simulink model "UAV_SIMULATOR_CA_2021a"  (R2024a)
settings: Solver=FixedStepAuto  StartTime=0.0  StopTime=tf_echelons  FixedStep=0.002  RelTol=1e-4
values from neighbouring files (symbols this model uses):
  Beta_OPT = [Beta, Z_max: 0.1*pi/180: betaf]    [UAV_SIMULATOR_MAIN_0.m]
  betaf = 20*pi/180 +betai    (= 0.660268528005)    [UAV_SIMULATOR_MAIN_0.m]
  betai = 17.8306*pi/180    (= 0.311202677606)    [UAV_SIMULATOR_MAIN_0.m]
  Bp_offset = 0.06    [UAV_SIMULATOR_MAIN_0.m]
  CDy = data(1)    [Aero_initial.m]    (also in FunLagragian.m; UAV_SIMULATOR_MAIN_0.m = 1; costFunction.m; nonLinearConstraints.m)
  CLOSED_LOOP_ESCs = 1    [UAV_SIMULATOR_MAIN_0.m]
  cQ = 2.1113*1e-08    (= 2.1113e-08)    [UAV_SIMULATOR_MAIN_0.m]
  cQ_Magnus = 0.5*S/2*RM^3*Cf    (= 4.804078125e-10)    [UAV_SIMULATOR_MAIN_0.m]
  cT = 2.4815e-6    (= 2.4815e-06)    [UAV_SIMULATOR_MAIN_0.m]
  cT_1_6 = 2.1030e-06    (= 2.103e-06)    [UAV_SIMULATOR_MAIN_0.m]
  D_PQR_PX4 = diag([D_ROLL D_PITCH D_YAW])    [UAV_SIMULATOR_MAIN_0.m]
  ethaf = 25*pi/180    (= 0.436332312999)    [UAV_SIMULATOR_MAIN_0.m]
  ethai = 0 *pi/180    (= 0)    [UAV_SIMULATOR_MAIN_0.m]
  F_fric = 0.5    [UAV_SIMULATOR_MAIN_0.m]
  Fa_L_int = Rmat*(FaG_int+FaG_int_d)    [UAV_SIMULATOR_MAIN_0.m]
  g = data(7)    [FunLagragian.m]    (also in UAV_SIMULATOR_MAIN_0.m = 9.81; costFunction.m; nonLinearConstraints.m; runOptimizationHelper.m = comp(7))
  I_PQR_PX4 = diag([I_ROLL I_PITCH I_YAW])    [UAV_SIMULATOR_MAIN_0.m]
  initial_attitude_condition = 1*[0 0 pi]    [UAV_SIMULATOR_MAIN_0.m]
  initial_pos_conditions = [ri*cos(betai) 0 ri*sin(betai) + Bp_offset]    [UAV_SIMULATOR_MAIN_0.m]
  Jr = 1.2991*1e-05    (= 1.2991e-05)    [UAV_SIMULATOR_MAIN_0.m]
  Jr_Magnus = JM1(2,2)    [UAV_SIMULATOR_MAIN_0.m]
  K_DI_int = [diag([k_r(1), k_etha(1), k_beta(1)]), diag([k_r(2), k_etha(2), k_beta(2)]), diag([k_r(3), k_etha(3), k_beta(3)])]    [UAV_SIMULATOR_MAIN_0.m]
  K_PQR_PX4 = 1*diag([0.8 1.35 1])    [UAV_SIMULATOR_MAIN_0.m]
  km = 1/Kv_motor_rad    (= 0.00545674090601)    [UAV_SIMULATOR_MAIN_0.m]
  L = lqr(A,B,Q_beta,R_beta)    [UAV_SIMULATOR_MAIN_0.m]
  L_mot = 1.0000e-04    (= 0.0001)    [UAV_SIMULATOR_MAIN_0.m]
  LM = 0.28*2    (= 0.56)    [UAV_SIMULATOR_MAIN_0.m]
  m = data(6)    [FunLagragian.m]    (also in UAV_SIMULATOR_MAIN_0.m = 1.746; costFunction.m; nonLinearConstraints.m; runOptimizationHelper.m = comp(6))
  m_M1 = 0.049    [UAV_SIMULATOR_MAIN_0.m]
  m_M2 = 0.049    [UAV_SIMULATOR_MAIN_0.m]
  m_w = 0.0481    [UAV_SIMULATOR_MAIN_0.m]    (also in nonLinearConstraints.m = data(9); runOptimizationHelper.m = comp(9))
  max_angle = max_angle_deg*pi/180    (= 0.610865238198)    [UAV_SIMULATOR_MAIN_0.m]
  nb_battery_cells = 4    [UAV_SIMULATOR_MAIN_0.m]
  P_ATTITUDE_PX4 = diag([10 10 2.8])    [UAV_SIMULATOR_MAIN_0.m]
  P_PQR_PX4 = diag([P_ROLL P_PITCH P_YAW])    [UAV_SIMULATOR_MAIN_0.m]
  PX4_attitude_loop_frequency = 250    [UAV_SIMULATOR_MAIN_0.m]
  PX4_rate_loop_frequency = 500    [UAV_SIMULATOR_MAIN_0.m]
  R = data(4)    [Aero_initial.m]    (also in UAV_SIMULATOR_MAIN_0.m = 0.07)
  R_bat = 0.024    [UAV_SIMULATOR_MAIN_0.m]
  rf = 1.5    [UAV_SIMULATOR_MAIN_0.m]
  rho_air = data(8)    [FunLagragian.m]    (also in UAV_SIMULATOR_MAIN_0.m = 1.293; costFunction.m; nonLinearConstraints.m; runOptimizationHelper.m = comp(8))
  ri = 0.490142    [UAV_SIMULATOR_MAIN_0.m]
  RM = data(4)    [FunLagragian.m]    (also in UAV_SIMULATOR_MAIN_0.m = 0.0275; costFunction.m; nonLinearConstraints.m; runOptimizationHelper.m = comp(4))
  S = data(3)    [Aero_initial.m]    (also in FunLagragian.m; UAV_SIMULATOR_MAIN_0.m = 0.0308; costFunction.m; nonLinearConstraints.m)
  s_M1D = [0, LM/4, 0]'    [UAV_SIMULATOR_MAIN_0.m]
  s_M2D = [0, -LM/4, 0]'    [UAV_SIMULATOR_MAIN_0.m]
  Slat = data(2)    [Aero_initial.m]    (also in FunLagragian.m; UAV_SIMULATOR_MAIN_0.m = 0.00237582944428; costFunction.m; nonLinearConstraints.m)
  state_int = [0 0 0 initial_attitude_condition 0 0 0 initial_attitude_quaternion_condition]    [UAV_SIMULATOR_MAIN_0.m]
  T0 = 1.5    [UAV_SIMULATOR_MAIN_0.m]
  t0 = 0    [UAV_SIMULATOR_MAIN_0.m]
  t1 = t0 + 15    (= 15)    [UAV_SIMULATOR_MAIN_0.m]
  t1T = t1/10    (= 1.5)    [UAV_SIMULATOR_MAIN_0.m]
  t2 = t1 + 15    (= 30)    [UAV_SIMULATOR_MAIN_0.m]    (also in plot_test.m = Simulation_Data.time)
  t2T = t2 + 9*t1/10    (= 43.5)    [UAV_SIMULATOR_MAIN_0.m]
  t3 = t2 + 15    (= 45)    [UAV_SIMULATOR_MAIN_0.m]
  tau_ur_model = 0.001    [UAV_SIMULATOR_MAIN_0.m]
  Tf = 1.5    [UAV_SIMULATOR_MAIN_0.m]
  Ti = 0    [UAV_SIMULATOR_MAIN_0.m]
  Ts = 0.02    [UAV_SIMULATOR_MAIN_0.m]
  U_sat = 3.7*nb_battery_cells    (= 14.8)    [UAV_SIMULATOR_MAIN_0.m]
  ViconTracker_noise_mean = 0.00001    (= 1e-05)    [UAV_SIMULATOR_MAIN_0.m]
  ViconTracker_noise_variance = 0.000001    (= 1e-06)    [UAV_SIMULATOR_MAIN_0.m]
  vitesse_vent = [0, 0, 0]'    [UAV_SIMULATOR_MAIN_0.m]
  vmag = 0    [UAV_SIMULATOR_MAIN_0.m]
  vx_wind = [vwind(1,1:t_winddirc_change/dt-1) vx_inter vwind(1,(t_winddirc_change+1)/dt +1:final_time/dt+1)*cos(10*pi/180)]    [UAV_SIMULATOR_MAIN_0.m]
  vy_wind = [zeros(1,t_winddirc_change/dt-1) vy_inter vwind(1,(t_winddirc_change+1)/dt +1:final_time/dt+1)*sin(10*pi/180)]    [UAV_SIMULATOR_MAIN_0.m]
  wind_turb = 1    [UAV_SIMULATOR_MAIN_0.m]
  wn_beta = 2    [UAV_SIMULATOR_MAIN_0.m]
  wn_etha = 2    [UAV_SIMULATOR_MAIN_0.m]
  wn_r = 2    [UAV_SIMULATOR_MAIN_0.m]
  X0 = 4    [UAV_SIMULATOR_MAIN_0.m]    (also in runOptimizationHelper.m = data(19))
  X1 = min(X1,8)    [Aero_initial.m]    (also in UAV_SIMULATOR_MAIN_0.m = [X1, X1(end)])
undefined symbols (not defined in the file or in its folder): DiscIntNeverNeededParam, PWM_data_map
libraries: simulink x23, slpidlib x5, eeGeneralControl x3, simulink_extras x1
(part 3 of 3)

== system UAV_SIMULATOR_CA_2021a/X4 + PX4 /X4 ESC PWM [OPEN LOOP MOTOR]1/Subsystem4/Subsystem2 ==
  In1 : Inport
  Gain4 : Gain  Gain=km
  Gain5 : Gain  Gain=km
  Gain6 : Gain  Gain=0.000001
  Gain7 : Gain  Gain=cQ
  Product1 : Product
  Sum3 : Sum  Inputs=|+-
  Sum4 : Sum  Inputs=-|+|-
  Transfer Fcn2 : TransferFcn  Denominator=[L_mot R]
  Transfer Fcn3 : TransferFcn  Denominator=[Jr 0]
  Out1 : Outport  VectorParamsAs1DForOutWhenUnconnected=off
  Out2 : Outport  Port=2  VectorParamsAs1DForOutWhenUnconnected=off
  wires:
  Sum4/1 -> Transfer Fcn3/1
  Gain5/1 -> Sum3/2  "FEM"
  Transfer Fcn3/1 -> Product1/2, Product1/1, Out1/1, Gain6/1, Gain5/1  "W"
  Gain4/1 -> Sum4/2  "Gama_mot"
  Product1/1 -> Gain7/1
  Gain6/1 -> Sum4/3  "Gamma_fric"
  Sum3/1 -> Transfer Fcn2/1
  Gain7/1 -> Sum4/1  "Gama_load"
  Transfer Fcn2/1 -> Out2/1, Gain4/1  "Motor_current"
  In1/1 -> Sum3/1  "U"

== system UAV_SIMULATOR_CA_2021a/X4 + PX4 /X4 ESC PWM [OPEN LOOP MOTOR]1/Subsystem4/Subsystem3 ==
  In1 : Inport
  Gain4 : Gain  Gain=km
  Gain5 : Gain  Gain=km
  Gain6 : Gain  Gain=0.000001
  Gain7 : Gain  Gain=cQ
  Product1 : Product
  Sum3 : Sum  Inputs=|+-
  Sum4 : Sum  Inputs=-|+|-
  Transfer Fcn2 : TransferFcn  Denominator=[L_mot R]
  Transfer Fcn3 : TransferFcn  Denominator=[Jr 0]
  Out1 : Outport  VectorParamsAs1DForOutWhenUnconnected=off
  Out2 : Outport  Port=2  VectorParamsAs1DForOutWhenUnconnected=off
  wires:
  In1/1 -> Sum3/1  "U"
  Transfer Fcn2/1 -> Gain4/1, Out2/1  "Motor_current"
  Gain7/1 -> Sum4/1  "Gama_load"
  Sum3/1 -> Transfer Fcn2/1
  Gain6/1 -> Sum4/3  "Gamma_fric"
  Product1/1 -> Gain7/1
  Gain4/1 -> Sum4/2  "Gama_mot"
  Transfer Fcn3/1 -> Gain5/1, Gain6/1, Out1/1, Product1/1, Product1/2  "W"
  Gain5/1 -> Sum3/2  "FEM"
  Sum4/1 -> Transfer Fcn3/1

== matlab function UAV_SIMULATOR_CA_2021a/spherical coordinates/MATLAB Function ==
  data: input input; spher_coord output
function  spher_coord = cart2spher(input)
x = input(1);
y = input(2);
z = input(3);
x_dot = input(4);
y_dot = input(5);
z_dot = input(6);

r = sqrt(x^2+y^2+z^2); %length of tether, [m]
if r > 0
    r_dir = -[x,y,z]./r; %unit vector of the tether [3x1] in inertial frame {I}
else
    r_dir = -[0,0,1];
end

xy=sqrt(x^2+y^2);
if xy ~= 0
  beta = atan2(z,xy);
  beta_dot = (xy*z_dot-z*(x*x_dot+y*y_dot)/xy)/r^2;
  etha_dot = (x*y_dot-y*x_dot)/(xy^2);
else
    beta = pi/2;
    etha_dot = 0;
    beta_dot = 0;
end


etha = atan2(y,x);
if r ~= 0
 r_dot = (x*x_dot+y*y_dot+z*z_dot)/r;
else
    r_dot = 0;
    beta_dot = 0;
end

spher_coord = [r etha beta r_dot etha_dot beta_dot r_dir];
spher_coord = double(spher_coord);
end

== matlab function UAV_SIMULATOR_CA_2021a/MATLAB Function6 ==
  data: input input; uT0_prev output
function uT0_prev = fcn(input)
Td=input(1);
r=input(2);
etha=input(3);
beta=input(4);
phi=input(5);
theta=input(6);
psi=input(7);
uT0_prev=Td*(cos(etha)*cos(beta)*cos(phi)*sin(theta)*cos(psi)+cos(etha)*cos(beta)*sin(phi)*sin(psi)+sin(etha)*cos(beta)*cos(phi)*sin(theta)*sin(psi)-sin(etha)*cos(beta)*sin(phi)*cos(psi)+sin(beta)*cos(phi)*cos(theta));
end

== matlab function UAV_SIMULATOR_CA_2021a/Subsystem2/MATLAB Function2 ==
  data: x_e input; xdot_e output; control input; data input
function xdot_e  = model_ekf(x_e,control, data)   % state : x_e =(r,dr,beta,dbeta,L,D)
m_w = data(1); 
m   = data(2); 
g   = data(3);

ur    = control(1);
uT    = control(2);
ubeta = control(3);
uetha = control(4);

xdot_e = [x_e(2);
         (1/(m+m_w))*(x_e(1)*x_e(6)^2*m +x_e(1)*x_e(4)^2*cos(x_e(5))^2*m -ur -m*g*sin(x_e(5))+uT + x_e(7));
         x_e(4);
         (1/(x_e(1)*cos(x_e(5))))*(-2*x_e(2)*x_e(4)*cos(x_e(5))+2*x_e(1)*x_e(4)*x_e(6)*sin(x_e(5))+1/m*uetha+1/m*x_e(8));
         x_e(6);
         (1/x_e(1))*(-2*x_e(2)*x_e(6)-x_e(1)*x_e(4)^2*cos(x_e(5))*sin(x_e(5))-g*cos(x_e(5))+1/m*ubeta + 1/m*x_e(9)); 
         0;
         0;
         0];
end

== matlab function UAV_SIMULATOR_CA_2021a/Subsystem2/Noice on Covariance ==
  data: u input; y output
function y = fcn(u)
y=randn*1e-4;
end

== matlab function UAV_SIMULATOR_CA_2021a/MATLAB Function2 ==
  data: Fa_G input; Fa_L output; data input
function Fa_L = fcn(Fa_G, data)
eta=data(2);
beta=data(3);
R_GS = [cos(eta)*cos(beta) sin(eta)*cos(beta) sin(beta);
                -sin(eta) cos(eta) 0;
                 -cos(eta)*sin(beta) -sin(eta)*sin(beta) cos(beta)];
Fa_L = R_GS * Fa_G;
end

== matlab function UAV_SIMULATOR_CA_2021a/MATLAB Function1 ==
  data: FaL input; u output; x input; data input
function u= fcn(FaL,x,data)
m = data(1);
m_w = data(2);
A = [(-1)/(m+m_w) 0 0;
    0 1/(m*x(1)*cos(x(3))) 0;
    0 0 1/(m*x(1))];
u = A * FaL;
end

== matlab function UAV_SIMULATOR_CA_2021a/2D LF Control3/CA optimisation problem1 ==
  settings: updateMethod=DISCRETE
  data: data input; optimized_X output; F_res_spherical output; Fa_zLB output; fval output; exitflag output; gradient output
function [optimized_X, F_res_spherical, Fa_zLB, fval, exitflag, gradient] = calculateOptimizedMagnusAndResidualForces(data)
% Wrapper that calls the full optimization helper (executed in MATLAB interpreter)

coder.extrinsic('runOptimizationHelper')

% Predefine output sizes and types
optimized_X = 0;
F_res_spherical = zeros(3,1);
Fa_zLB = 0;
fval = 0;
exitflag = int8(0);
gradient = 0;

% Call helper that performs all optimization and aerodynamic calculations
[optimized_X, F_res_spherical, Fa_zLB, fval, exitflag, gradient] = runOptimizationHelper(data);
end

== matlab function UAV_SIMULATOR_CA_2021a/MATLAB Function3 ==
  data: Fa_G input; Fa_L output; data input
function Fa_L = fcn(Fa_G, data)
eta=data(2);
beta=data(3);
R_GS = [cos(eta)*cos(beta) sin(eta)*cos(beta) sin(beta);
                -sin(eta) cos(eta) 0;
                 -cos(eta)*sin(beta) -sin(eta)*sin(beta) cos(beta)];
Fa_L = R_GS * Fa_G;
end

== matlab function UAV_SIMULATOR_CA_2021a/2D LF Control3/Compensation of F_res 1 ==
  data: pos_spherical input; F_res_spherical input; Fa_zLB input; thrust_ref output; phi_ref output; psi input; theta_ref output; psi_vicon input
function [thrust_ref, phi_ref, theta_ref] = calculateThrustAndPhi(pos_spherical, F_res_spherical, Fa_zLB, psi,psi_vicon)
    

    r    = pos_spherical(1);
    etha = pos_spherical(2);
    beta = pos_spherical(3);

    delta_FT    = F_res_spherical(1);
    delta_Feta  = F_res_spherical(2);
    delta_Fbeta = F_res_spherical(3);

    thrust_ref = norm(F_res_spherical);
    
    theta_ref = atan2((delta_FT*cos(etha)*cos(beta) - delta_Feta*sin(etha) - delta_Fbeta*cos(etha)*sin(beta)) * cos(psi+psi_vicon) +...
        (delta_FT*sin(etha)*cos(beta) + delta_Feta*cos(etha) - delta_Fbeta*sin(etha)*sin(beta)) * sin(psi+psi_vicon), (delta_FT*sin(beta) + delta_Fbeta*cos(beta)));

    T_dy = thrust_ref + Fa_zLB;%force acting on y direction
    if T_dy == 0  
      phi_ref = 0;
    else
      phi_ref = asin(((-delta_FT*sin(etha)*cos(beta) - delta_Feta*cos(etha) + delta_Fbeta*sin(etha)*sin(beta)) *cos(psi+psi_vicon) + ...
          (delta_FT*cos(etha)*cos(beta) - delta_Feta*sin(etha) - delta_Fbeta*cos(etha)*sin(beta)) * sin(psi+psi_vicon))/T_dy);
    end

%     theta_ref = atan2((delta_FT*cos(etha)*cos(beta) - delta_Feta*sin(etha) - delta_Fbeta*cos(etha)*sin(beta)) / cos(psi), (delta_FT*sin(beta) + delta_Fbeta*cos(beta)));
% 
%     T_dy = thrust_ref + Fa_zLB;%force acting on y direction
%     if T_dy == 0  
%       phi_ref = 0;
%     else
%       phi_ref = asin((-delta_FT*sin(etha)*cos(beta) - delta_Feta*cos(etha) + delta_Fbeta*sin(etha)*sin(beta)) /(T_dy*cos(psi)));
%     end
end

== matlab function UAV_SIMULATOR_CA_2021a/2D LF Control3/MATLAB Function ==
  data: input input; Va_G output
function Va_G = fcn(input)
V_wind = input(1:3);
V_system = input(4:6);
Va_G = V_wind - V_system;
end

== matlab function UAV_SIMULATOR_CA_2021a/2D LF Control3/MATLAB Function1 ==
  data: betaref input; BETA_OPT input; X1 input; X0 input; X_opt output
function X_opt  = fcn(betaref, BETA_OPT, X1, X0)
I=1;
while BETA_OPT(I)<=betaref && BETA_OPT(I)~=BETA_OPT(end)
    I=I+1;
end
X_opt=double(X1(I));
end

== matlab function UAV_SIMULATOR_CA_2021a/3D PID- open Loop uT/MATLAB Function ==
  data: input input; output output; psi input; max_roll_pitch input

function output = Thrust_phi_theta(input, psi, max_roll_pitch) 

Fx = input(1);
Fy = input(2);
Fz = input(3);


FX = cos(psi) * Fx  + sin(psi) * Fy;
FY = -sin(psi) * Fx + cos(psi) * Fy;


theta = atan2(FX,Fz);
if abs(theta) > max_roll_pitch
    theta = sign(theta) * max_roll_pitch;
    FX = Fz * tan(theta);
end
    
phi = atan2(-FY, sqrt(Fz^2+FX^2));
if abs(phi) > max_roll_pitch
   phi = sign(phi) * max_roll_pitch;
   FY = sqrt(Fz^2 + FX^2) * tan(phi);
end 
    

T_d = sqrt(FX^2 + FY^2 + Fz^2);  


T_ref = T_d;
phi_ref = phi;
theta_ref = theta;

output= [phi_ref,theta_ref, T_ref];
end

== matlab function UAV_SIMULATOR_CA_2021a/3D PID- open Loop uT/MATLAB Function1 ==
  settings: updateMethod=DISCRETE
  data: Trajectory_Error input; u_winch output; Integral_Error input; Derivative input; pos_speed_spher input; Feed_Forward input; data input; K_DI_int input; u_UAV output; data1 input; v output; ie_beta output; L input; T0 input; T_error input; T_error_int input
function [u_winch, u_UAV, v, ie_beta] = calculatePIDControlInput(Trajectory_Error,Integral_Error, Derivative, pos_speed_spher, Feed_Forward, data, K_DI_int,...
    data1, L, T0, T_error, T_error_int)

m_w = data(1);
wn_r = data(2);
wn_beta = data(3);
wn_etha = data(4);
m = data(5);    % mass of the total system
g = data(6);
%T0 = data(7);   % desired tether traction forc
betai = data(7); 
betaf = data(8);

v_beta_saturate_upper = 1.2;% m*g*cos(betai) + 0.1;
v_beta_saturate_lower = -0.1;% m*g*cos(max_angle) -0.1;


e_r    = Trajectory_Error(1);
e_etha = Trajectory_Error(2);
e_beta = Trajectory_Error(3);

de_r    = Trajectory_Error(4);
de_etha = Trajectory_Error(5);
de_beta = Trajectory_Error(6);

ie_r    = Integral_Error(1);
ie_etha = Integral_Error(2);
ie_beta = Integral_Error(3);

ddr    = Derivative(4);

r    = pos_speed_spher(1);
etha = pos_speed_spher(2);
beta = pos_speed_spher(3);

d_r    = pos_speed_spher(4);
d_etha = pos_speed_spher(5);
d_beta = pos_speed_spher(6);

% Feed Forward Terms
Fa_r    = Feed_Forward(1);
Fa_etha  = Feed_Forward(2);
Fa_beta = Feed_Forward(3);

if(r == 0)
    u_winch = 0;
    u_UAV = [0, 0, 0];
    v = [0, 0, 0]';
else
    
    
    %u_r_1 = 2*0.7*wn_r*de_r       + wn_r^2*e_r ;
    u_T = T0 + m*g*sin(beta);% + m*ddr;     % open loop on u_T 
   
    A = [-1/(m + m_w)      0               0;
            0       1/(m*r*cos(beta))      0;
            0              0            1/(m*r)];
        
    b=[(1/(m + m_w)) * ((r*d_beta^2 + r*d_etha^2*cos(beta)^2)*m - m*g*sin(beta) + u_T + Fa_r);
        
        (-2*d_r*d_etha*cos(beta) + 2*r*d_etha*d_beta*sin(beta) + (1/m) * Fa_etha)/(r*cos(beta));
        
        (-2*d_r*d_beta - r*d_etha^2*cos(beta)*sin(beta) - g*cos(beta) + (1/m)*Fa_beta)/r];

% Feedback Linearization based on PID + Anti windup 
    v_r    = 2.1396*wn_r*de_r       + 2.172*wn_r^2*e_r       + wn_r^3*ie_r;
    v_etha = 2.1396*wn_etha*de_etha  + 2.172*wn_etha^2*e_etha + wn_etha^3*ie_etha;
    v_beta = 2.1396*wn_beta*de_beta + 2.172*wn_beta^2*e_beta + wn_beta^3*ie_beta;
    
    
    % Feed back controller
    v=[v_r;v_etha;v_beta];
    u=A\(v-b);

    u_winch = u(1);
    %u_T = u_T + 1*max(1*(T0 - T) + 1*T_int,0);
    %u_T = u_T + 1*max(dT + 2*0.7*2*(T0 - T) + 2^2*T_int,0);
    %u_T = u_T +1 * max(1 * T_error, 0) + max(1 * T_error_int, 0);
    u_UAV = [u_T, u(2), u(3)];

end

== matlab function UAV_SIMULATOR_CA_2021a/3D PID- open Loop uT/MATLAB Function3 ==
  data: input input; pos_spher input; output output; psi_V input

function output = Thrust_phi_theta(input, pos_spher, psi_V) 

u_T    = input(1);
u_etha = input(2);
u_beta = input(3);

etha = pos_spher(2);
beta = pos_spher(3);

Fx = cos(etha)*cos(beta)*u_T - sin(etha)*u_etha -cos(etha)*sin(beta)*u_beta;
Fy = sin(etha)*cos(beta)*u_T + cos(etha)*u_etha -sin(etha)*sin(beta)*u_beta;
Fz = sin(beta)*u_T + cos(beta)*u_beta;
R = [cos(psi_V) sin(psi_V) 0; 
    -sin(psi_V) cos(psi_V) 0; 
          0         0      1];
      
output= R * [Fx, Fy, Fz]';
end

== matlab function UAV_SIMULATOR_CA_2021a/3D STSMC- CA uT/MATLAB Function ==
  data: input input; output output; psi input; max_roll_pitch input

function output = Thrust_phi_theta(input, psi, max_roll_pitch) 

Fx = input(1);
Fy = input(2);
Fz = input(3);


FX = cos(psi) * Fx  + sin(psi) * Fy;
FY = -sin(psi) * Fx + cos(psi) * Fy;


theta = atan2(FX,Fz);
if abs(theta) > max_roll_pitch
    theta = sign(theta) * max_roll_pitch;
    FX = Fz * tan(theta);
end
    
phi = atan2(-FY, sqrt(Fz^2+FX^2));
if abs(phi) > max_roll_pitch
   phi = sign(phi) * max_roll_pitch;
   FY = sqrt(Fz^2 + FX^2) * tan(phi);
end 
    

T_d = sqrt(FX^2 + FY^2 + Fz^2);  


T_ref = T_d;
phi_ref = phi;
theta_ref = theta;

output= [phi_ref,theta_ref, T_ref];
end

== matlab function UAV_SIMULATOR_CA_2021a/3D STSMC- CA uT/MATLAB Function1 ==
  settings: updateMethod=DISCRETE
  data: Trajectory_Error input; u_winch output; Integral_Error input; pos_speed_dot input; pos_speed_spher input; Feed_Forward input; data input; u_UAV output; S_SMC output; T0 input; dwfunc output; wfunc input; K1 input; K2 input; Psi input; dK1 output; dK2 output
function [u_winch, u_UAV, S_SMC, dwfunc, dK1, dK2] = calculatePIDControlInput(Trajectory_Error,Integral_Error, pos_speed_dot, pos_speed_spher, Feed_Forward, data, T0, wfunc, K1, K2, Psi)

m_w = data(1);
lmr = data(2);
lmb = data(3);
lme = data(4);
m = data(5);    % mass of the total system
g = data(6);

wr=wfunc(1);
we=wfunc(2);
wb=wfunc(3);

e_r    = Trajectory_Error(1);
e_etha = Trajectory_Error(2);
e_beta = Trajectory_Error(3);

de_r    = Trajectory_Error(4);
de_etha = Trajectory_Error(5);
de_beta = Trajectory_Error(6);

ie_r    = Integral_Error(1);
ie_etha = Integral_Error(2);
ie_beta = Integral_Error(3);


r    = pos_speed_spher(1);
etha = pos_speed_spher(2);
beta = pos_speed_spher(3);

d_r    = pos_speed_spher(4);
d_etha = pos_speed_spher(5);
d_beta = pos_speed_spher(6);

% Feed Forward Terms
Fa_r    = Feed_Forward(1);
Fa_etha  = Feed_Forward(2);
Fa_beta = Feed_Forward(3);

r_ddot = pos_speed_dot(4);

if(r == 0)
    u_winch = 0;
    u_UAV = [0, 0, 0]';
    S_SMC = [0, 0, 0]';
    dK1 = [0, 0, 0]';
    dK2 = [0, 0, 0]';
    dwfunc = [0, 0, 0]';
else
    
    u_T = T0 + m*g*sin(beta);     % open loop on u_T 
   
    A = [-1/(m + m_w)      0               0;
            0       1/(m*r*cos(beta))      0;
            0              0            1/(m*r)];
        
    b=[(1/(m + m_w)) * ((r*d_beta^2 + r*d_etha^2*cos(beta)^2)*m - m*g*sin(beta) + u_T + Fa_r);
        
        (-2*d_r*d_etha*cos(beta) + 2*r*d_etha*d_beta*sin(beta) + (1/m) * Fa_etha)/(r*cos(beta));
        
        (-2*d_r*d_beta - r*d_etha^2*cos(beta)*sin(beta) - g*cos(beta) + (1/m)*Fa_beta)/r];


% Feedback Linearization based on PID + Anti windup 
%     kr1 = K1(1);
%     ke1 = K1(2);
%     kb1 = K1(3);
%     
%     kr2 = K2(1);
%     ke2 = K2(2);
%     kb2 = K2(3);

    psi_r = Psi(1);
    psi_e = Psi(2);
    psi_b = Psi(3);
    
    epsilon_r = 0.1;
    epsilon_e = 0.1;
    epsilon_b = 0.1;
    
    alpha_r = 2.5;%1.5;
    alpha_e = 1;%0.8;
    alpha_b = 2;%1.3;
    
    kr1 = 4;
    ke1 = 1.5;
    kb1 = 4.5;
    
    kr2 = 1.1*kr1;
    ke2 = 1.1*ke1;
    kb2 = 1.1*kb1;
    
    lmr = 1.5;
    lme = 1.6;
    lmb = 1.5;
   
    
    Sr = - de_r    - lmr*e_r;
    Se = - de_etha - lme*e_etha;
    Sb = - de_beta - lmb*e_beta;
    
    v_r    = 2*lmr * de_r    - kr1*sqrt(abs(Sr))*tanh(Sr/0.3) + wr;
    %v_etha = 2*lme * de_etha - ke1*sqrt(abs(Se))*tanh(Se/0.2) + we;
    v_beta = 2*lmb * de_beta - kb1*sqrt(abs(Sb))*tanh(Sb/0.3) + wb;
    
    %v_r    = 2*lmr * de_r + lmr^2*e_r   - kr1*sqrt(abs(Sr))*tanh(Sr/0.3) + wr;
    v_etha = 2*lme * de_etha + lme^2*e_etha  - ke1*sqrt(abs(Se))*tanh(Se/0.3) + we;
    %v_beta = 2*lmb * de_beta + lmb^2*e_beta - kb1*sqrt(abs(Sb))*tanh(Sb/0.3) + wb;
   

    dwr=-kr2 * tanh(Sr/0.3);
    dwe=-ke2 * tanh(Se/0.3);
    dwb=-kb2 * tanh(Sb/0.3);
    dwfunc=[dwr;dwe;dwb];

    % Feed back controller
    v=[v_r;v_etha;v_beta];
    u=A\(v-b);

    u_winch = u(1);
    u_UAV = [u_T, u(2), u(3)]';

    S_SMC = [Sr, Se, Sb]';
    
    if abs(Sr) <= epsilon_r
        dkr1 = -kr1;
        dkr2 = -kr2;
       
    else
        dkr1 = alpha_r/ (psi_r + epsilon_r);
        dkr2 = alpha_r/(2*sqrt(abs(Sr)));
    end
    
    if abs(Se) <= epsilon_e
        dke1 = -ke1;
        dke2 = -ke2;
    else
        dke1 = alpha_e/ (psi_e + epsilon_e);
        dke2 = alpha_e/(2*sqrt(abs(Se)));
    end
    
    if abs(Sb) <= epsilon_b
        dkb1 = -kb1;
        dkb2 = -kb2;
    else
        dkb1 = alpha_b/ (psi_b + epsilon_b);
        dkb2 = alpha_b/(2*sqrt(abs(Sb)));
    end
        
    dK1 = [dkr1, dke1, dkb1]';
    dK2 = [dkr2, dke2, dkb2]';
end

== matlab function UAV_SIMULATOR_CA_2021a/X4 + PX4 /X4 ESC PWM [OPEN LOOP MOTOR]1/MATLAB Function2 ==
  data: Fa_G input; Fa_L output; data input
function Fa_L = fcn(Fa_G, data)
eta=data(2);
beta=data(3);
R_GS = [cos(eta)*cos(beta) sin(eta)*cos(beta) sin(beta);
                -sin(eta) cos(eta) 0;
                 -cos(eta)*sin(beta) -sin(eta)*sin(beta) cos(beta)];

Fa_L = R_GS * Fa_G;

end

== matlab function UAV_SIMULATOR_CA_2021a/3D STSMC- CA uT/MATLAB Function3 ==
  data: input input; pos_spher input; output output; psi_V input

function output = Thrust_phi_theta(input, pos_spher, psi_V) 

u_T    = input(1);
u_etha = input(2);
u_beta = input(3);

etha = pos_spher(2);
beta = pos_spher(3);

Fx = cos(etha)*cos(beta)*u_T - sin(etha)*u_etha -cos(etha)*sin(beta)*u_beta;
Fy = sin(etha)*cos(beta)*u_T + cos(etha)*u_etha -sin(etha)*sin(beta)*u_beta;
Fz = sin(beta)*u_T + cos(beta)*u_beta;
R = [cos(psi_V) sin(psi_V) 0; 
    -sin(psi_V) cos(psi_V) 0; 
          0         0      1];
      
output= R * [Fx, Fy, Fz]';
end

== matlab function UAV_SIMULATOR_CA_2021a/MATLAB Function7 ==
  data: Fa_L input; Fa_G output; data input
function Fa_G = fcn(Fa_L, data)
eta=data(2);
beta=data(3);
R_GS = [cos(eta)*cos(beta) sin(eta)*cos(beta) sin(beta);
                -sin(eta) cos(eta) 0;
                 -cos(eta)*sin(beta) -sin(eta)*sin(beta) cos(beta)];
Fa_G = inv(R_GS) * Fa_L';
end

== matlab function UAV_SIMULATOR_CA_2021a/Winch Model/Bridle Point Torque ==
  data: Tension_Force input; Torque_bridlepoint output; lcb input; spher_coord input; quad input; Tension_body output
function [Torque_bridlepoint, Tension_body] = fcn(Tension_Force, lcb, spher_coord, quad)
eta = spher_coord(2); 
beta = spher_coord(3);
q0 = quad(1); q1 = quad(2); q2 = quad(3); q3 = quad(4); 
R_GL = inv([(q0^2 + q1^2 - q2^2 - q3^2)  2*(q1*q2 - q0*q3) 2*(q1*q3 + q0*q2) ;
                 2*(q1*q2 + q0*q3)  (q0^2 - q1^2 + q2^2 - q3^2) 2*(q2*q3 - q0*q1) ;
                 2*(q1*q3 - q0*q2) 2*(q2*q3 + q0*q1) (q0^2 - q1^2 - q2^2 + q3^2) ] );
Tension_body = R_GL*Tension_Force;
Torque_bridlepoint = -cross(lcb, Tension_body);
end

== matlab function UAV_SIMULATOR_CA_2021a/spherical coordinates/MATLAB Function1 ==
  data: in1 input; y output
function y = fcn(in1)
q0=in1(1);
q1=in1(2);
q2=in1(3);
q3=in1(4);


y = [(q0^2 + q1^2 - q2^2 - q3^2)  2*(q1*q2 - q0*q3) 2*(q1*q3 + q0*q2) ;
                 2*(q1*q2 + q0*q3)  (q0^2 - q1^2 + q2^2 - q3^2) 2*(q2*q3 - q0*q1) ;
                 2*(q1*q3 - q0*q2) 2*(q2*q3 + q0*q1) (q0^2 - q1^2 - q2^2 + q3^2) ] ;
     
end

== matlab function UAV_SIMULATOR_CA_2021a/Control Inputs in Spher ==
  data: data input; Fa_pher output
function Fa_pher = fcn(data)

Thrust = data(1);
r = data(2); eta=data(3); beta = data(4);
quaternions = data(5:8);
q0 = quaternions(1) ;
q1 = quaternions(2) ;
q2 = quaternions(3) ;
q3 = quaternions(4) ;

Fa_L = [0; 0; Thrust];

R_LG = [(q0^2 + q1^2 - q2^2 - q3^2)  2*(q1*q2 - q0*q3) 2*(q1*q3 + q0*q2) ;
                 2*(q1*q2 + q0*q3)  (q0^2 - q1^2 + q2^2 - q3^2) 2*(q2*q3 - q0*q1) ;
                 2*(q1*q3 - q0*q2) 2*(q2*q3 + q0*q1) (q0^2 - q1^2 - q2^2 + q3^2) ] ;
             
Fa_G = R_LG * Fa_L;

R_GS = [cos(eta)*cos(beta) sin(eta)*cos(beta) sin(beta);
                -sin(eta) cos(eta) 0;
                 -cos(eta)*sin(beta) -sin(eta)*sin(beta) cos(beta)];
             
Fa_pher = R_GS * Fa_G;
end

== matlab function UAV_SIMULATOR_CA_2021a/MATLAB Function ==
  data: X input; w_ref output; Va input; RM input
function w_ref = fcn(X,Va,RM)
Vaxz=norm([Va(1) 0 Va(3)]);
w_ref=(X*Vaxz/RM);
% if w<4000
%     w_ref=4000*(2*pi/60);
% else 
%     w_ref=(X*Vaxz/RM);
% end

== matlab function UAV_SIMULATOR_CA_2021a/Aerodynamic Forces/MATLAB Function ==
  data: Va input; Va_r input; Va_l input; data input; Fa_LB output; wmag input; quad input; Fa_G output; Gamma output; s_M1D input; s_M2D input
function [Fa_LB,Fa_G,Gamma] = fcn(Va, Va_r, Va_l, data, wmag, quad, s_M1D, s_M2D)

CDy=data(1);
Slat=data(2);
S=data(3);
R=data(4);
L=data(5);
m_M1=data(6);
m_M2=data(7);
m=data(8);
rho_air = data(9);

% Error on lift and right wind on Magnus cylinders due to nonhomegneous of wind speed distrbution because of the 
% wind tunnel 

model_error_r = 1;%0.7; 
model_error_l = 1;

%Error on the Magnus Aerodynamics
model_error = 1;

q0=quad(1);q1=quad(2);q2=quad(3);q3=quad(4);
R_matrix = [(q0^2 + q1^2 - q2^2 - q3^2)  2*(q1*q2 - q0*q3) 2*(q1*q3 + q0*q2) ;
                 2*(q1*q2 + q0*q3)  (q0^2 - q1^2 + q2^2 - q3^2) 2*(q2*q3 - q0*q1) ;
                 2*(q1*q3 - q0*q2) 2*(q2*q3 + q0*q1) (q0^2 - q1^2 - q2^2 + q3^2) ] ;            
             

s_CD=(m_M1*s_M1D'+m_M2*s_M2D')/m;
s_DC=-s_CD;
s_MrC=s_M1D'+s_DC;
s_MlC=s_M2D'+s_DC;

%%right Magnus            
Va=Va_r*model_error_r;
F_a_r_y_local = (1/2)*CDy*Slat*abs(Va(2))*Va(2);
Vaxz=norm([Va(1) Va(3)]);
if Vaxz==0
     eFD=[1 0 0];
     X1=0;
else
     eFD=[Va(1)/Vaxz 0 Va(3)/Vaxz];
     X1= min(wmag*R/Vaxz,7);%saturation car validité du modele à X=<7
     %X1= wmag*R/Vaxz;
end
eFL=cross([0 1 0],eFD);
X1  = min(X1,8);

CL = ((1 - 1./(1 + exp(-0.904 * X1))).*(0.0276*X1^4+4.6595*X1^3-6.0369*X1^2+2.9557*X1) +  1./(1 + exp(-0.904 * X1)) .*(1.0849*X1))*model_error;
CD = (-0.0461 * X1^3 + 0.5167 * X1^2 -0.6511 * X1 +0.9081)*model_error;


F_L_r_xz_local = (1/2)*rho_air*CL*S/2*Vaxz^2*eFL;
F_D_r_xz_local = (1/2)*rho_air*CD*S/2*Vaxz^2*eFD;
Fa_r_LB = [0 F_a_r_y_local 0]+F_D_r_xz_local+F_L_r_xz_local;
Gamma_right=cross(s_MrC,Fa_r_LB')+[0 0.5*S/2*R^3*0.003*wmag^2 0];


%%lift Magnus
Va=Va_l*model_error_l;
F_a_l_y_local = (1/2)*CDy*Slat*abs(Va(2))*Va(2);
Vaxz=norm([Va(1) Va(3)]);
if Vaxz==0
     eFD=[1 0 0];
     X1=0;
else
     eFD=[Va(1)/Vaxz 0 Va(3)/Vaxz];
     X1= min(wmag*R/Vaxz,7);%saturation car validité du modele à X=<7
end
eFL=cross([0 1 0],eFD);
X1  = min(X1,8);

CL = ((1 - 1./(1 + exp(-0.904 * X1))).*(0.0276*X1^4+4.6595*X1^3-6.0369*X1^2+2.9557*X1) +  1./(1 + exp(-0.904 * X1)) .*(1.0849*X1)) * model_error;
CD = (-0.0461 * X1^3 + 0.5167 * X1^2 -0.6511 * X1 +0.9081)* model_error;

F_L_l_xz_local = (1/2)*rho_air*CL*S/2*Vaxz^2*eFL;
F_D_l_xz_local = (1/2)*rho_air*CD*S/2*Vaxz^2*eFD;
Fa_l_LB = [0 F_a_l_y_local 0]+F_D_l_xz_local+F_L_l_xz_local;
Gamma_lift=cross(s_MlC,Fa_l_LB')+[0 0.5*S/2*R^3*0.003*wmag^2 0];

Fa_LB=Fa_r_LB+Fa_l_LB;
Fa_G1=R_matrix*Fa_LB';
Fa_G=Fa_G1;
Gamma=Gamma_right+Gamma_lift;
end

== matlab function UAV_SIMULATOR_CA_2021a/Aerodynamic Forces/MATLAB Function1 ==
  data: input input; Va output; Va_r output; Va_l output
function [Va,Va_r,Va_l]= App_wind_lr(input)
vx_wind = input(1);
vy_wind = input(2);
vz_wind = input(3);
vx = input(4);
vy = input(5);
vz = input(6);
q0 = input(7) ; 
q1 = input(8) ;
q2 = input(9) ;
q3 = input(10) ;
r=input(13);
l=input(14);
R_matrix = [(q0^2 + q1^2 - q2^2 - q3^2)  2*(q1*q2 - q0*q3) 2*(q1*q3 + q0*q2) ;
                 2*(q1*q2 + q0*q3)  (q0^2 - q1^2 + q2^2 - q3^2) 2*(q2*q3 - q0*q1) ;
                 2*(q1*q3 - q0*q2) 2*(q2*q3 + q0*q1) (q0^2 - q1^2 - q2^2 + q3^2) ] ;
Va_inertial=[vx_wind-vx vy_wind-vy vz_wind-vz]';
Va_local= R_matrix\Va_inertial;
Va=[Va_local(1) Va_local(2) Va_local(3)];
Va_r=[Va(1)+r*l/4 0 Va(3)];
Va_l=[Va(1)-r*l/4 0 Va(3)];
end

== matlab function UAV_SIMULATOR_CA_2021a/MATLAB Function5 ==
  data: input input; ub_prev output
function ub_prev = fcn(input)
Td=input(1);
r=input(2);
etha=input(3);
beta=input(4);
phi=input(5);
theta=input(6);
psi=input(7);
ub_prev=Td*(-sin(beta)*cos(etha)*cos(phi)*sin(theta)*cos(psi)+sin(beta)*sin(etha)*sin(phi)*cos(psi)+cos(beta)*cos(phi)*cos(theta));
ub_prev=ub_prev+Td*(-sin(beta)*cos(theta)*sin(phi)*sin(psi)-sin(beta)*sin(theta)*cos(phi)*sin(theta)*sin(psi));
end

== matlab function UAV_SIMULATOR_CA_2021a/MATLAB Function4 ==
  data: input input; ue_prev output
function ue_prev = fcn(input)
Td=input(1);
r=input(2);
etha=input(3);
beta=input(4);
phi=input(5);
theta=input(6);
psi=input(7);
ue_prev=Td*(-sin(etha)*cos(phi)*sin(theta)*cos(psi)-cos(etha)*sin(phi)*cos(psi));
ue_prev=ue_prev+Td*(-sin(etha)*sin(phi)*sin(psi)+cos(etha)*cos(phi)*sin(theta)*sin(psi));
end

== matlab function UAV_SIMULATOR_CA_2021a/Subsystem2/MATLAB Function1 ==
  data: y input; x_est output; pos_updated input; speed input; Cov input; Thrust input; euler_angles input; Cov1 output; data input
function [x_est,Cov1] = Kalman(y, pos_updated, speed, Cov, Thrust, euler_angles, data) 

m_w = data(1); 
m   = data(2); 
g   = data(3); 
Ts  = data(4);

q1=1e-10; q2=20;  q3=q1; q4=q2; q5=q1; q6=q2; q7=80; q8=q7; q9=q7; q=[q1;q2;q3;q4;q5;q6;q7;q8;q9]; Q=diag(q); %How we trust our mathematical model 
r1=1e-10; r2=r1; r3=r1; r=[r1;r2;r3]; R=diag(r); %measurment noice covariance matrix, could be obtained from sensor datasheet

% if xupdated==zeros(9,1)
%     xupdated=[0.5*cos(20*pi/180); 0 ;0 ; 0; 0.5*sin(20*pi/180);0;0;0;0];
% end

h = @(x) [x(1); x(3); x(5)];
F = f_jacobian(pos_updated, Thrust, euler_angles, m, m_w, g);
A = eye(9) + Ts * F;
H = [1 0 0 0 0 0 0 0 0; 0 0 1 0 0 0 0 0 0; 0 0 0 0 1 0 0 0 0];  

xpredict = pos_updated + Ts * speed; % la discretisation du modèle non linéaire 
ypredict = h(xpredict);

if Cov==0
    cov=eye(9);
else 
    cov=Cov;
end

cov = A * cov * A' + Q;
S   = H * cov * H' + R;   
Kf  = cov * H' / S; % Kalman Gain

pos_updated = xpredict + Kf * (y - ypredict);
yupdated = h(pos_updated); % Updating/correctin measurement
x_est = pos_updated;

Cov_up = (eye(9) - Kf * H) * cov; % Updating Covariance Matrix
Cov1   = Cov_up; % Overwriting covariance matrix

end
